simulink model "HW2_5_antiwindup"  (R2025b)
settings: Solver=VariableStepAuto  StartTime=0.0  StopTime=15  RelTol=1e-3
settings Model: Creator=BCC  LastModifiedBy=BCC

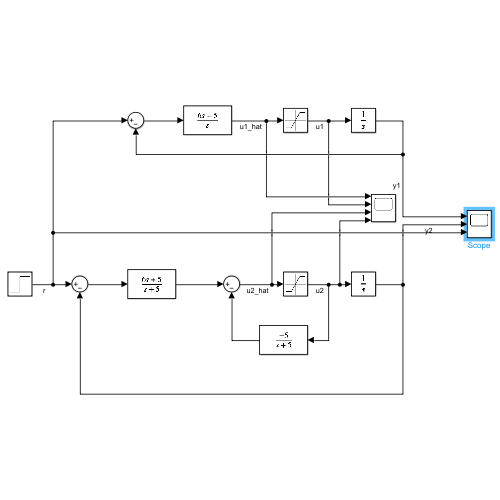
[thumbnail: Simulink's stored preview of the top-level diagram]
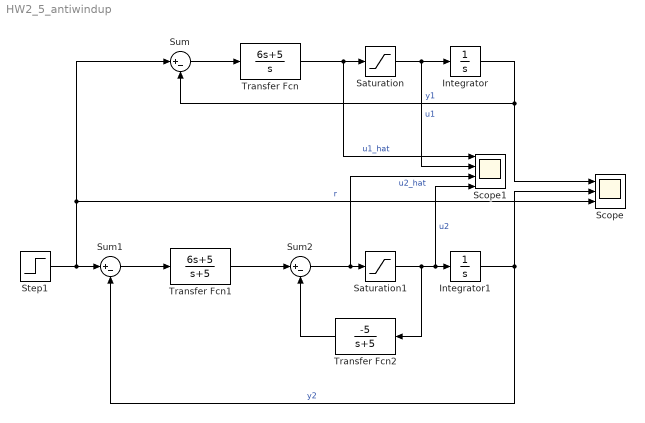
== system HW2_5_antiwindup ==
  Integrator : Integrator
  Integrator1 : Integrator
  Saturation : Saturate  UpperLimit=1  LowerLimit=-1
  Saturation1 : Saturate  UpperLimit=1  LowerLimit=-1
  Scope : Scope  NumInputPorts=3
      settings: ActiveDisplayYMinimum=-0.8659941860137641  ActiveDisplayYMaximum=7.7939476741238787
  Scope1 : Scope  NumInputPorts=4
      settings: ActiveDisplayYMinimum=-14.769368056981481  ActiveDisplayYMaximum=50.02392506982391
  Step1 : Step  After=4  SampleTime=0
  Sum : Sum  Inputs=|+-
  Sum1 : Sum  Inputs=|+-
  Sum2 : Sum  Inputs=|+-
  Transfer Fcn : TransferFcn  Numerator=[6 5]  Denominator=[1 0]
  Transfer Fcn1 : TransferFcn  Numerator=[6 5]  Denominator=[1 5]
  Transfer Fcn2 : TransferFcn  Numerator=[-5]  Denominator=[1 5]
  wires:
  Transfer Fcn/1 -> Scope1/1, Saturation/1  "u1_hat"
  Integrator/1 -> Sum/2, Scope/1  "y1"
  Saturation/1 -> Scope1/2, Integrator/1  "u1"
  Step1/1 -> Scope/3, Sum/1, Sum1/1  "r"
  Sum/1 -> Transfer Fcn/1
  Integrator1/1 -> Scope/2, Sum1/2  "y2"
  Sum1/1 -> Transfer Fcn1/1
  Saturation1/1 -> Scope1/4, Integrator1/1, Transfer Fcn2/1  "u2"
  Transfer Fcn2/1 -> Sum2/2
  Transfer Fcn1/1 -> Sum2/1
  Sum2/1 -> Scope1/3, Saturation1/1  "u2_hat"
